simulink library "casper_library_correlator"  (Simulink 8.0)
settings: Solver=ode45  SolverMode=SingleTasking  StartTime=0.0  StopTime=10.0  RelTol=1e-3
values from neighbouring files (symbols this model uses):
  n_bits = eval(get_var('n_bits', 'defaults', defaults, varargin{:}))    [auto_tap_init.m]    (also in baseline_tap_init.m; bi_real_unscr_2x_init.m = get_var('n_bits', 'defaults', defaults, varargin{:}); bi_real_unscr_4x_init.m = get_var('n_bits', 'defaults', defaults, varargin{:}); bit_reverse_init.m = get_var('n_bits',varargin{:}))
libraries: xbsIndex_r4 x1360, casper_library_misc x140, casper_library_multipliers x32, xps_library x8, casper_library_delays x1, casper_library_correlator x1
(part 10 of 14)

== system casper_library_correlator/auto_tap/dual_pol_cmac/cmac1/cmult* ==
  a : Inport
  b : Inport  Port=2
  a_expand : Subsystem  AncestorBlock=casper_library_flow_control/bus_expand  mask(bus_expand){mode=divisions of equal size, outputNum=4, outputWidth=[4 4 4 4], outputBinaryPt=[3 3 3 3], outputArithmeticType=[1 1 1 1], show_format=off, outputToWorkspace=off, variablePrefix=out, outputToModelAsWell=on}
      mask prompts: outputNum "Number of outputs:"; outputWidth "Output width:"; outputBinaryPt "Output binary point position:"; outputArithmeticType "Output arithmetic type (ufix=0, fix=1, bool=2):"; show_format "Print format string?"; outputToWorkspace "Output to workspace?"; variablePrefix "Variable name prefix:"; outputToModelAsWell "Output to model as well?"
      mask help:
      | Expands a 'bus' made using a bus_create or Xilinx
      | concat block.
      | The input will be divided into the specified number
      | of outputs with the specified arithmetic types.
      | Divisions are made from most significant bit.
      mask init: same as casper_library_correlator/dual_pol_cmac/cmac1/cmult*/a_expand
      settings: AttributesFormatString=4 outputs
      mask TypeOptions mode: divisions of equal size | divisions of arbitrary size
      mask Callback mode: bus_expand_callback();
      mask Callback outputWidth: bus_expand_callback();
      mask Callback outputToWorkspace: bus_expand_callback();
  a_replicate : Subsystem  AncestorBlock=casper_library_bus/bus_replicate  mask(bus_replicate){replication=2, latency=0, misc=off, implementation=core}
      mask prompts: replication "replication factor"; misc "misc support"; implementation "delay implementation"
      mask help: Output bus formed by replicating input bus a number of times
      mask init:
      | bus_replicate_init(gcb, ...
      |     'replication', replication, ...
      |     'latency', latency, ...
      |     'implementation', implementation, ...
      |     'misc', misc);
      mask TypeOptions implementation: core | behavioral
  addsub_im : xbsIndex_r4/AddSub  mode=Subtraction  use_carryin=off  use_carryout=off  en=off  latency=1  precision=Full  arith_type=Unsigned  n_bits=16  bin_pt=14  quantization=Truncate  overflow=Wrap  dbl_ovrd=off  use_behavioral_HDL=on  hw_selection=Fabric  pipelined=on  use_rpm=on  block_type=addsub
  addsub_re : xbsIndex_r4/AddSub  mode=Addition  use_carryin=off  use_carryout=off  en=off  latency=1  precision=Full  arith_type=Unsigned  n_bits=16  bin_pt=14  quantization=Truncate  overflow=Wrap  dbl_ovrd=off  use_behavioral_HDL=on  hw_selection=Fabric  pipelined=on  use_rpm=on  block_type=addsub
  b_expand : Subsystem  AncestorBlock=casper_library_flow_control/bus_expand  mask(bus_expand){mode=divisions of equal size, outputNum=4, outputWidth=[4 4 4 4], outputBinaryPt=[3 3 3 3], outputArithmeticType=[1 1 1 1], show_format=off, outputToWorkspace=off, variablePrefix=out, outputToModelAsWell=on}
      mask prompts: outputNum "Number of outputs:"; outputWidth "Output width:"; outputBinaryPt "Output binary point position:"; outputArithmeticType "Output arithmetic type (ufix=0, fix=1, bool=2):"; show_format "Print format string?"; outputToWorkspace "Output to workspace?"; variablePrefix "Variable name prefix:"; outputToModelAsWell "Output to model as well?"
      mask help:
      | Expands a 'bus' made using a bus_create or Xilinx
      | concat block.
      | The input will be divided into the specified number
      | of outputs with the specified arithmetic types.
      | Divisions are made from most significant bit.
      mask init: same as casper_library_correlator/dual_pol_cmac/cmac1/cmult*/a_expand
      settings: AttributesFormatString=4 outputs
      mask TypeOptions mode: divisions of equal size | divisions of arbitrary size
      mask Callback mode: bus_expand_callback();
      mask Callback outputWidth: bus_expand_callback();
      mask Callback outputToWorkspace: bus_expand_callback();
  b_replicate : Subsystem  AncestorBlock=casper_library_bus/bus_replicate  mask(bus_replicate){replication=2, latency=0, misc=off, implementation=core}
      mask prompts: replication "replication factor"; misc "misc support"; implementation "delay implementation"
      mask help: Output bus formed by replicating input bus a number of times
      mask init:
      | bus_replicate_init(gcb, ...
      |     'replication', replication, ...
      |     'latency', latency, ...
      |     'implementation', implementation, ...
      |     'misc', misc);
      mask TypeOptions implementation: core | behavioral
  convert_im : xbsIndex_r4/Convert  gui_display_data_type=Fixed-point  arith_type="Signed  (2's comp)"  n_bits=16  bin_pt=6  float_type=Single  exp_bits=8  fraction_bits=24  quantization=Truncate  overflow=Wrap  en=off  latency=0  dbl_ovrd=off  pipeline=on  block_type=convert
  convert_re : xbsIndex_r4/Convert  gui_display_data_type=Fixed-point  arith_type="Signed  (2's comp)"  n_bits=16  bin_pt=6  float_type=Single  exp_bits=8  fraction_bits=24  quantization=Truncate  overflow=Wrap  en=off  latency=0  dbl_ovrd=off  pipeline=on  block_type=convert
  imim : xbsIndex_r4/Mult  precision=Full  arith_type="Signed  (2's comp)"  n_bits=16  bin_pt=14  quantization=Truncate  overflow=Wrap  en=off  latency=1  dbl_ovrd=off  use_behavioral_HDL=off  opt=Speed  use_embedded=on  optimum_pipeline=off  pipeline=on  use_rpm=on  placement_style=Triangular  block_type=mult
  imre : xbsIndex_r4/Mult  precision=Full  arith_type="Signed  (2's comp)"  n_bits=16  bin_pt=14  quantization=Truncate  overflow=Wrap  en=off  latency=1  dbl_ovrd=off  use_behavioral_HDL=off  opt=Speed  use_embedded=on  optimum_pipeline=off  pipeline=on  use_rpm=on  placement_style=Triangular  block_type=mult
  reim : xbsIndex_r4/Mult  precision=Full  arith_type="Signed  (2's comp)"  n_bits=16  bin_pt=14  quantization=Truncate  overflow=Wrap  en=off  latency=1  dbl_ovrd=off  use_behavioral_HDL=off  opt=Speed  use_embedded=on  optimum_pipeline=off  pipeline=on  use_rpm=on  placement_style=Triangular  block_type=mult
  rere : xbsIndex_r4/Mult  precision=Full  arith_type="Signed  (2's comp)"  n_bits=16  bin_pt=14  quantization=Truncate  overflow=Wrap  en=off  latency=1  dbl_ovrd=off  use_behavioral_HDL=off  opt=Speed  use_embedded=on  optimum_pipeline=off  pipeline=on  use_rpm=on  placement_style=Triangular  block_type=mult
  ri_to_c : casper_library_misc/ri_to_c
  ab : Outport
  wires:
  ri_to_c/1 -> ab/1
  convert_im/1 -> ri_to_c/2
  convert_re/1 -> ri_to_c/1
  addsub_im/1 -> convert_im/1
  addsub_re/1 -> convert_re/1
  reim/1 -> addsub_im/2
  imre/1 -> addsub_im/1
  imim/1 -> addsub_re/2
  rere/1 -> addsub_re/1
  b_expand/4(lsb_out1) -> reim/2
  a_expand/3(out2) -> reim/1
  b_expand/3(out2) -> imre/2
  a_expand/4(lsb_out1) -> imre/1
  b_expand/2(out3) -> imim/2
  a_expand/2(out3) -> imim/1
  b_expand/1(msb_out4) -> rere/2
  a_expand/1(msb_out4) -> rere/1
  b_replicate/1(out) -> b_expand/1(bus_in)
  a_replicate/1(out) -> a_expand/1(bus_in)
  b/1 -> b_replicate/1(in)
  a/1 -> a_replicate/1(in)

== system casper_library_correlator/auto_tap/dual_pol_cmac/cmac1/ri_to_c ==
  In1 : Inport
  In2 : Inport  Port=2
  Concat : xbsIndex_r4/Concat  num_inputs=2  dbl_ovrd=off  block_type=concat
      settings: block_version=9.2.01
  Reinterpret : xbsIndex_r4/Reinterpret  force_arith_type=on  arith_type=Unsigned  force_bin_pt=on  bin_pt=0  block_type=reinterpret
      settings: infoedit="Changes signal type without altering the binary representation.   You can changed the signal between signed and unsigned, and relocate the binary point.<P><P>Hardware notes: In hardware this block costs nothing.<P><P>Example:  Suppose the input is 6 bits wide, signed, with 2 fractional bits, and the output is forced to unsigned with 0 fractional bits.  Then an input of -2.0 (1110.00 in binary 2's complement) becomes an output of 56 (111000 in binary)."  block_version=9.2.01
  Reinterpret1 : xbsIndex_r4/Reinterpret  force_arith_type=on  arith_type=Unsigned  force_bin_pt=on  bin_pt=0  block_type=reinterpret
      settings: infoedit="Changes signal type without altering the binary representation.   You can changed the signal between signed and unsigned, and relocate the binary point.<P><P>Hardware notes: In hardware this block costs nothing.<P><P>Example:  Suppose the input is 6 bits wide, signed, with 2 fractional bits, and the output is forced to unsigned with 0 fractional bits.  Then an input of -2.0 (1110.00 in binary 2's complement) becomes an output of 56 (111000 in binary)."  block_version=9.2.01
  Out1 : Outport
  wires:
  In2/1 -> Reinterpret1/1
  Concat/1 -> Out1/1
  In1/1 -> Reinterpret/1
  Reinterpret1/1 -> Concat/2
  Reinterpret/1 -> Concat/1

== system casper_library_correlator/auto_tap/dual_pol_cmac/cmac2/acc ==
  rst : Inport
  din : Inport  Port=2
  acc_in : Inport  Port=3
  valid_in : Inport  Port=4
  Accumulator : xbsIndex_r4/Accumulator  operation=Add  n_bits=n_bits_out  overflow=Wrap  scale=1  rst=on  infoeditControl=reset for floating point data type must be asserted for a minimum of 2 cycles  hasbypass=on  en=off  latency=0  dbl_ovrd=off  msb_inp=100  msb=100  lsb=-100  use_behavioral_HDL=on  implementation=Fabric  block_type=accum
      settings: infoedit="Adder or subtractor-based accumulator.   Output type and binary point position match the input.<P><P>Hardware notes: When \"Reinitialize with input 'b' on reset\" is selected, the accumulator is forced to run at the system rate even if the input 'b' is running at a slower rate."  xl_area=[0, 0, 0, 0, 0, 0, 0]  block_version=9.2.01
  Constant : xbsIndex_r4/Constant  const=1  gui_display_data_type=Fixed-point  arith_type=Boolean  n_bits=1  bin_pt=0  preci_type=Single  exp_width=8  frac_width=24  explicit_period=on  period=1  equ=P=C  opselect=C  inp2=PCIN>>17  opr=+  inp1=P  carry=CIN  dbl_ovrd=off  block_type=constant
      settings: block_version=9.2.01
  Convert1 : xbsIndex_r4/Convert  gui_display_data_type=Fixed-point  arith_type="Signed  (2's comp)"  n_bits=n_bits_out  bin_pt=bin_pt_out  float_type=Single  exp_bits=8  fraction_bits=24  quantization=Truncate  overflow=Wrap  en=off  latency=0  dbl_ovrd=off  pipeline=off  block_type=convert
      settings: xl_area=[0, 0, 0, 0, 0, 0, 0]  block_version=9.2.01
  Convert2 : xbsIndex_r4/Convert  gui_display_data_type=Fixed-point  arith_type=Boolean  n_bits=8  bin_pt=6  float_type=Single  exp_bits=8  fraction_bits=24  quantization=Truncate  overflow=Wrap  en=off  latency=0  dbl_ovrd=off  pipeline=off  block_type=convert
      settings: xl_area=[0, 0, 0, 0, 0, 0, 0]  block_version=9.2.01
  Delay : xbsIndex_r4/Delay  rst=off  infoeditControl=Selection of Reset will increase slice count due to use of real FFs and instead of SRLs  en=off  latency=0  dbl_ovrd=off  reg_retiming=off  block_type=delay
      settings: xl_area=[0, 0, 0, 0, 0, 0, 0]  block_version=9.2.01
  Delay1 : xbsIndex_r4/Delay  rst=off  infoeditControl=Selection of Reset will increase slice count due to use of real FFs and instead of SRLs  en=off  latency=0  dbl_ovrd=off  reg_retiming=off  block_type=delay
      settings: xl_area=[0, 0, 0, 0, 0, 0, 0]  block_version=9.2.01
  Mux2 : xbsIndex_r4/Mux  inputs=2  en=off  latency=2  precision=Full  arith_type="Signed  (2's comp)"  n_bits=0  bin_pt=0  quantization="Round  (unbiased: +/- Inf)"  overflow=Wrap  dbl_ovrd=off  block_type=mux
      settings: xl_area=[0, 0, 0, 0, 0, 0, 0]  block_version=9.2.01
  Mux3 : xbsIndex_r4/Mux  inputs=2  en=off  latency=2  precision=Full  arith_type="Signed  (2's comp)"  n_bits=0  bin_pt=0  quantization=Truncate  overflow=Wrap  dbl_ovrd=off  block_type=mux
      settings: xl_area=[0, 0, 0, 0, 0, 0, 0]  block_version=9.2.01
  acc_out : Outport
  valid_out : Outport  Port=2
  wires:
  Convert2/1 -> Mux3/2
  Delay1/1 -> Delay/1, Accumulator/2
  Convert1/1 -> Accumulator/1
  Delay/1 -> Mux2/1, Mux3/1
  rst/1 -> Delay1/1
  din/1 -> Convert1/1
  Mux3/1 -> valid_out/1
  Constant/1 -> Mux3/3
  valid_in/1 -> Convert2/1
  acc_in/1 -> Mux2/2
  Mux2/1 -> acc_out/1
  Accumulator/1 -> Mux2/3

== system casper_library_correlator/auto_tap/dual_pol_cmac/cmac2/acc1 ==
  rst : Inport
  din : Inport  Port=2
  acc_in : Inport  Port=3
  valid_in : Inport  Port=4
  Accumulator : xbsIndex_r4/Accumulator  operation=Add  n_bits=n_bits_out  overflow=Wrap  scale=1  rst=on  infoeditControl=reset for floating point data type must be asserted for a minimum of 2 cycles  hasbypass=on  en=off  latency=0  dbl_ovrd=off  msb_inp=100  msb=100  lsb=-100  use_behavioral_HDL=on  implementation=Fabric  block_type=accum
      settings: infoedit="Adder or subtractor-based accumulator.   Output type and binary point position match the input.<P><P>Hardware notes: When \"Reinitialize with input 'b' on reset\" is selected, the accumulator is forced to run at the system rate even if the input 'b' is running at a slower rate."  xl_area=[0, 0, 0, 0, 0, 0, 0]  block_version=9.2.01
  Constant : xbsIndex_r4/Constant  const=1  gui_display_data_type=Fixed-point  arith_type=Boolean  n_bits=1  bin_pt=0  preci_type=Single  exp_width=8  frac_width=24  explicit_period=on  period=1  equ=P=C  opselect=C  inp2=PCIN>>17  opr=+  inp1=P  carry=CIN  dbl_ovrd=off  block_type=constant
      settings: block_version=9.2.01
  Convert1 : xbsIndex_r4/Convert  gui_display_data_type=Fixed-point  arith_type="Signed  (2's comp)"  n_bits=n_bits_out  bin_pt=bin_pt_out  float_type=Single  exp_bits=8  fraction_bits=24  quantization=Truncate  overflow=Wrap  en=off  latency=0  dbl_ovrd=off  pipeline=off  block_type=convert
      settings: xl_area=[0, 0, 0, 0, 0, 0, 0]  block_version=9.2.01
  Convert2 : xbsIndex_r4/Convert  gui_display_data_type=Fixed-point  arith_type=Boolean  n_bits=8  bin_pt=6  float_type=Single  exp_bits=8  fraction_bits=24  quantization=Truncate  overflow=Wrap  en=off  latency=0  dbl_ovrd=off  pipeline=off  block_type=convert
      settings: xl_area=[0, 0, 0, 0, 0, 0, 0]  block_version=9.2.01
  Delay : xbsIndex_r4/Delay  rst=off  infoeditControl=Selection of Reset will increase slice count due to use of real FFs and instead of SRLs  en=off  latency=0  dbl_ovrd=off  reg_retiming=off  block_type=delay
      settings: xl_area=[0, 0, 0, 0, 0, 0, 0]  block_version=9.2.01
  Delay1 : xbsIndex_r4/Delay  rst=off  infoeditControl=Selection of Reset will increase slice count due to use of real FFs and instead of SRLs  en=off  latency=0  dbl_ovrd=off  reg_retiming=off  block_type=delay
      settings: xl_area=[0, 0, 0, 0, 0, 0, 0]  block_version=9.2.01
  Mux2 : xbsIndex_r4/Mux  inputs=2  en=off  latency=2  precision=Full  arith_type="Signed  (2's comp)"  n_bits=0  bin_pt=0  quantization="Round  (unbiased: +/- Inf)"  overflow=Wrap  dbl_ovrd=off  block_type=mux
      settings: xl_area=[0, 0, 0, 0, 0, 0, 0]  block_version=9.2.01
  Mux3 : xbsIndex_r4/Mux  inputs=2  en=off  latency=2  precision=Full  arith_type="Signed  (2's comp)"  n_bits=0  bin_pt=0  quantization=Truncate  overflow=Wrap  dbl_ovrd=off  block_type=mux
      settings: xl_area=[0, 0, 0, 0, 0, 0, 0]  block_version=9.2.01
  acc_out : Outport
  valid_out : Outport  Port=2
  wires:
  Accumulator/1 -> Mux2/3
  Mux2/1 -> acc_out/1
  acc_in/1 -> Mux2/2
  valid_in/1 -> Convert2/1
  Constant/1 -> Mux3/3
  Mux3/1 -> valid_out/1
  din/1 -> Convert1/1
  rst/1 -> Delay1/1
  Delay/1 -> Mux3/1, Mux2/1
  Convert1/1 -> Accumulator/1
  Delay1/1 -> Accumulator/2, Delay/1
  Convert2/1 -> Mux3/2

== system casper_library_correlator/auto_tap/dual_pol_cmac/cmac2/c_to_ri1 ==
  In1 : Inport
  Reinterpret : xbsIndex_r4/Reinterpret  force_arith_type=on  arith_type="Signed  (2's comp)"  force_bin_pt=on  bin_pt=bin_pt_out  block_type=reinterpret
      settings: block_version=9.2.01
  Reinterpret1 : xbsIndex_r4/Reinterpret  force_arith_type=on  arith_type="Signed  (2's comp)"  force_bin_pt=on  bin_pt=bin_pt_out  block_type=reinterpret
      settings: block_version=9.2.01
  Slice : xbsIndex_r4/Slice  nbits=n_bits_out  boolean_output=off  mode=Upper Bit Location + Width  bit1=0  base1=MSB of Input  bit0=0  base0=LSB of Input  dbl_ovrd=off  block_type=slice
      settings: infoedit="Extracts a given range of bits from each input sample and presents it at the output.  The output type is ordinarily unsigned with binary point at zero, but can be Boolean when the slice is one bit wide.<P><P>Hardware notes: In hardware this block costs nothing."  block_version=9.2.01
  Slice1 : xbsIndex_r4/Slice  nbits=n_bits_out  boolean_output=off  mode=Lower Bit Location + Width  bit1=0  base1=MSB of Input  bit0=0  base0=LSB of Input  dbl_ovrd=off  block_type=slice
      settings: infoedit="Extracts a given range of bits from each input sample and presents it at the output.  The output type is ordinarily unsigned with binary point at zero, but can be Boolean when the slice is one bit wide.<P><P>Hardware notes: In hardware this block costs nothing."  block_version=9.2.01
  Out1 : Outport
  Out2 : Outport  Port=2
  wires:
  In1/1 -> Slice1/1, Slice/1
  Reinterpret1/1 -> Out2/1
  Reinterpret/1 -> Out1/1
  Slice1/1 -> Reinterpret1/1
  Slice/1 -> Reinterpret/1

== system casper_library_correlator/auto_tap/dual_pol_cmac/cmac2/c_to_ri2 ==
  In1 : Inport
  Reinterpret : xbsIndex_r4/Reinterpret  force_arith_type=on  arith_type="Signed  (2's comp)"  force_bin_pt=on  bin_pt=n_bits_out - bit_growth - 3  block_type=reinterpret
      settings: infoedit="Changes signal type without altering the binary representation.   You can changed the signal between signed and unsigned, and relocate the binary point.<P><P>Hardware notes: In hardware this block costs nothing.<P><P>Example:  Suppose the input is 6 bits wide, signed, with 2 fractional bits, and the output is forced to unsigned with 0 fractional bits.  Then an input of -2.0 (1110.00 in binary 2's complement) becomes an output of 56 (111000 in binary)."  block_version=9.2.01
  Reinterpret1 : xbsIndex_r4/Reinterpret  force_arith_type=on  arith_type="Signed  (2's comp)"  force_bin_pt=on  bin_pt=n_bits_out - bit_growth - 3  block_type=reinterpret
      settings: infoedit="Changes signal type without altering the binary representation.   You can changed the signal between signed and unsigned, and relocate the binary point.<P><P>Hardware notes: In hardware this block costs nothing.<P><P>Example:  Suppose the input is 6 bits wide, signed, with 2 fractional bits, and the output is forced to unsigned with 0 fractional bits.  Then an input of -2.0 (1110.00 in binary 2's complement) becomes an output of 56 (111000 in binary)."  block_version=9.2.01
  Slice : xbsIndex_r4/Slice  nbits=n_bits_out  boolean_output=off  mode=Upper Bit Location + Width  bit1=0  base1=MSB of Input  bit0=0  base0=LSB of Input  dbl_ovrd=off  block_type=slice
      settings: infoedit="Extracts a given range of bits from each input sample and presents it at the output.  The output type is ordinarily unsigned with binary point at zero, but can be Boolean when the slice is one bit wide.<P><P>Hardware notes: In hardware this block costs nothing."  block_version=9.2.01
  Slice1 : xbsIndex_r4/Slice  nbits=n_bits_out  boolean_output=off  mode=Lower Bit Location + Width  bit1=0  base1=MSB of Input  bit0=0  base0=LSB of Input  dbl_ovrd=off  block_type=slice
      settings: infoedit="Extracts a given range of bits from each input sample and presents it at the output.  The output type is ordinarily unsigned with binary point at zero, but can be Boolean when the slice is one bit wide.<P><P>Hardware notes: In hardware this block costs nothing."  block_version=9.2.01
  Out1 : Outport
  Out2 : Outport  Port=2
  wires:
  Slice/1 -> Reinterpret/1
  Slice1/1 -> Reinterpret1/1
  Reinterpret/1 -> Out1/1
  Reinterpret1/1 -> Out2/1
  In1/1 -> Slice/1, Slice1/1

== system casper_library_correlator/auto_tap/dual_pol_cmac/cmac2/cmult* ==
  a : Inport
  b : Inport  Port=2
  a_expand : Subsystem  AncestorBlock=casper_library_flow_control/bus_expand  mask(bus_expand){mode=divisions of equal size, outputNum=4, outputWidth=[4 4 4 4], outputBinaryPt=[3 3 3 3], outputArithmeticType=[1 1 1 1], show_format=off, outputToWorkspace=off, variablePrefix=out, outputToModelAsWell=on}
      mask prompts: outputNum "Number of outputs:"; outputWidth "Output width:"; outputBinaryPt "Output binary point position:"; outputArithmeticType "Output arithmetic type (ufix=0, fix=1, bool=2):"; show_format "Print format string?"; outputToWorkspace "Output to workspace?"; variablePrefix "Variable name prefix:"; outputToModelAsWell "Output to model as well?"
      mask help:
      | Expands a 'bus' made using a bus_create or Xilinx
      | concat block.
      | The input will be divided into the specified number
      | of outputs with the specified arithmetic types.
      | Divisions are made from most significant bit.
      mask init: same as casper_library_correlator/dual_pol_cmac/cmac1/cmult*/a_expand
      settings: AttributesFormatString=4 outputs
      mask TypeOptions mode: divisions of equal size | divisions of arbitrary size
      mask Callback mode: bus_expand_callback();
      mask Callback outputWidth: bus_expand_callback();
      mask Callback outputToWorkspace: bus_expand_callback();
  a_replicate : Subsystem  AncestorBlock=casper_library_bus/bus_replicate  mask(bus_replicate){replication=2, latency=0, misc=off, implementation=core}
      mask prompts: replication "replication factor"; misc "misc support"; implementation "delay implementation"
      mask help: Output bus formed by replicating input bus a number of times
      mask init:
      | bus_replicate_init(gcb, ...
      |     'replication', replication, ...
      |     'latency', latency, ...
      |     'implementation', implementation, ...
      |     'misc', misc);
      mask TypeOptions implementation: core | behavioral
  addsub_im : xbsIndex_r4/AddSub  mode=Subtraction  use_carryin=off  use_carryout=off  en=off  latency=1  precision=Full  arith_type=Unsigned  n_bits=16  bin_pt=14  quantization=Truncate  overflow=Wrap  dbl_ovrd=off  use_behavioral_HDL=on  hw_selection=Fabric  pipelined=on  use_rpm=on  block_type=addsub
  addsub_re : xbsIndex_r4/AddSub  mode=Addition  use_carryin=off  use_carryout=off  en=off  latency=1  precision=Full  arith_type=Unsigned  n_bits=16  bin_pt=14  quantization=Truncate  overflow=Wrap  dbl_ovrd=off  use_behavioral_HDL=on  hw_selection=Fabric  pipelined=on  use_rpm=on  block_type=addsub
  b_expand : Subsystem  AncestorBlock=casper_library_flow_control/bus_expand  mask(bus_expand){mode=divisions of equal size, outputNum=4, outputWidth=[4 4 4 4], outputBinaryPt=[3 3 3 3], outputArithmeticType=[1 1 1 1], show_format=off, outputToWorkspace=off, variablePrefix=out, outputToModelAsWell=on}
      mask prompts: outputNum "Number of outputs:"; outputWidth "Output width:"; outputBinaryPt "Output binary point position:"; outputArithmeticType "Output arithmetic type (ufix=0, fix=1, bool=2):"; show_format "Print format string?"; outputToWorkspace "Output to workspace?"; variablePrefix "Variable name prefix:"; outputToModelAsWell "Output to model as well?"
      mask help:
      | Expands a 'bus' made using a bus_create or Xilinx
      | concat block.
      | The input will be divided into the specified number
      | of outputs with the specified arithmetic types.
      | Divisions are made from most significant bit.
      mask init: same as casper_library_correlator/dual_pol_cmac/cmac1/cmult*/a_expand
      settings: AttributesFormatString=4 outputs
      mask TypeOptions mode: divisions of equal size | divisions of arbitrary size
      mask Callback mode: bus_expand_callback();
      mask Callback outputWidth: bus_expand_callback();
      mask Callback outputToWorkspace: bus_expand_callback();
  b_replicate : Subsystem  AncestorBlock=casper_library_bus/bus_replicate  mask(bus_replicate){replication=2, latency=0, misc=off, implementation=core}
      mask prompts: replication "replication factor"; misc "misc support"; implementation "delay implementation"
      mask help: Output bus formed by replicating input bus a number of times
      mask init:
      | bus_replicate_init(gcb, ...
      |     'replication', replication, ...
      |     'latency', latency, ...
      |     'implementation', implementation, ...
      |     'misc', misc);
      mask TypeOptions implementation: core | behavioral
  convert_im : xbsIndex_r4/Convert  gui_display_data_type=Fixed-point  arith_type="Signed  (2's comp)"  n_bits=16  bin_pt=6  float_type=Single  exp_bits=8  fraction_bits=24  quantization=Truncate  overflow=Wrap  en=off  latency=0  dbl_ovrd=off  pipeline=on  block_type=convert
  convert_re : xbsIndex_r4/Convert  gui_display_data_type=Fixed-point  arith_type="Signed  (2's comp)"  n_bits=16  bin_pt=6  float_type=Single  exp_bits=8  fraction_bits=24  quantization=Truncate  overflow=Wrap  en=off  latency=0  dbl_ovrd=off  pipeline=on  block_type=convert
  imim : xbsIndex_r4/Mult  precision=Full  arith_type="Signed  (2's comp)"  n_bits=16  bin_pt=14  quantization=Truncate  overflow=Wrap  en=off  latency=1  dbl_ovrd=off  use_behavioral_HDL=off  opt=Speed  use_embedded=on  optimum_pipeline=off  pipeline=on  use_rpm=on  placement_style=Triangular  block_type=mult
  imre : xbsIndex_r4/Mult  precision=Full  arith_type="Signed  (2's comp)"  n_bits=16  bin_pt=14  quantization=Truncate  overflow=Wrap  en=off  latency=1  dbl_ovrd=off  use_behavioral_HDL=off  opt=Speed  use_embedded=on  optimum_pipeline=off  pipeline=on  use_rpm=on  placement_style=Triangular  block_type=mult
  reim : xbsIndex_r4/Mult  precision=Full  arith_type="Signed  (2's comp)"  n_bits=16  bin_pt=14  quantization=Truncate  overflow=Wrap  en=off  latency=1  dbl_ovrd=off  use_behavioral_HDL=off  opt=Speed  use_embedded=on  optimum_pipeline=off  pipeline=on  use_rpm=on  placement_style=Triangular  block_type=mult
  rere : xbsIndex_r4/Mult  precision=Full  arith_type="Signed  (2's comp)"  n_bits=16  bin_pt=14  quantization=Truncate  overflow=Wrap  en=off  latency=1  dbl_ovrd=off  use_behavioral_HDL=off  opt=Speed  use_embedded=on  optimum_pipeline=off  pipeline=on  use_rpm=on  placement_style=Triangular  block_type=mult
  ri_to_c : casper_library_misc/ri_to_c
  ab : Outport
  wires:
  ri_to_c/1 -> ab/1
  convert_im/1 -> ri_to_c/2
  convert_re/1 -> ri_to_c/1
  addsub_im/1 -> convert_im/1
  addsub_re/1 -> convert_re/1
  reim/1 -> addsub_im/2
  imre/1 -> addsub_im/1
  imim/1 -> addsub_re/2
  rere/1 -> addsub_re/1
  b_expand/4(lsb_out1) -> reim/2
  a_expand/3(out2) -> reim/1
  b_expand/3(out2) -> imre/2
  a_expand/4(lsb_out1) -> imre/1
  b_expand/2(out3) -> imim/2
  a_expand/2(out3) -> imim/1
  b_expand/1(msb_out4) -> rere/2
  a_expand/1(msb_out4) -> rere/1
  b_replicate/1(out) -> b_expand/1(bus_in)
  a_replicate/1(out) -> a_expand/1(bus_in)
  b/1 -> b_replicate/1(in)
  a/1 -> a_replicate/1(in)

== system casper_library_correlator/auto_tap/dual_pol_cmac/cmac2/ri_to_c ==
  In1 : Inport
  In2 : Inport  Port=2
  Concat : xbsIndex_r4/Concat  num_inputs=2  dbl_ovrd=off  block_type=concat
      settings: block_version=9.2.01
  Reinterpret : xbsIndex_r4/Reinterpret  force_arith_type=on  arith_type=Unsigned  force_bin_pt=on  bin_pt=0  block_type=reinterpret
      settings: infoedit="Changes signal type without altering the binary representation.   You can changed the signal between signed and unsigned, and relocate the binary point.<P><P>Hardware notes: In hardware this block costs nothing.<P><P>Example:  Suppose the input is 6 bits wide, signed, with 2 fractional bits, and the output is forced to unsigned with 0 fractional bits.  Then an input of -2.0 (1110.00 in binary 2's complement) becomes an output of 56 (111000 in binary)."  block_version=9.2.01
  Reinterpret1 : xbsIndex_r4/Reinterpret  force_arith_type=on  arith_type=Unsigned  force_bin_pt=on  bin_pt=0  block_type=reinterpret
      settings: infoedit="Changes signal type without altering the binary representation.   You can changed the signal between signed and unsigned, and relocate the binary point.<P><P>Hardware notes: In hardware this block costs nothing.<P><P>Example:  Suppose the input is 6 bits wide, signed, with 2 fractional bits, and the output is forced to unsigned with 0 fractional bits.  Then an input of -2.0 (1110.00 in binary 2's complement) becomes an output of 56 (111000 in binary)."  block_version=9.2.01
  Out1 : Outport
  wires:
  In2/1 -> Reinterpret1/1
  Concat/1 -> Out1/1
  In1/1 -> Reinterpret/1
  Reinterpret1/1 -> Concat/2
  Reinterpret/1 -> Concat/1

== system casper_library_correlator/auto_tap/dual_pol_cmac/cmac3/acc ==
  rst : Inport
  din : Inport  Port=2
  acc_in : Inport  Port=3
  valid_in : Inport  Port=4
  Accumulator : xbsIndex_r4/Accumulator  operation=Add  n_bits=n_bits_out  overflow=Wrap  scale=1  rst=on  infoeditControl=reset for floating point data type must be asserted for a minimum of 2 cycles  hasbypass=on  en=off  latency=0  dbl_ovrd=off  msb_inp=100  msb=100  lsb=-100  use_behavioral_HDL=on  implementation=Fabric  block_type=accum
      settings: infoedit="Adder or subtractor-based accumulator.   Output type and binary point position match the input.<P><P>Hardware notes: When \"Reinitialize with input 'b' on reset\" is selected, the accumulator is forced to run at the system rate even if the input 'b' is running at a slower rate."  xl_area=[0, 0, 0, 0, 0, 0, 0]  block_version=9.2.01
  Constant : xbsIndex_r4/Constant  const=1  gui_display_data_type=Fixed-point  arith_type=Boolean  n_bits=1  bin_pt=0  preci_type=Single  exp_width=8  frac_width=24  explicit_period=on  period=1  equ=P=C  opselect=C  inp2=PCIN>>17  opr=+  inp1=P  carry=CIN  dbl_ovrd=off  block_type=constant
      settings: block_version=9.2.01
  Convert1 : xbsIndex_r4/Convert  gui_display_data_type=Fixed-point  arith_type="Signed  (2's comp)"  n_bits=n_bits_out  bin_pt=bin_pt_out  float_type=Single  exp_bits=8  fraction_bits=24  quantization=Truncate  overflow=Wrap  en=off  latency=0  dbl_ovrd=off  pipeline=off  block_type=convert
      settings: xl_area=[0, 0, 0, 0, 0, 0, 0]  block_version=9.2.01
  Convert2 : xbsIndex_r4/Convert  gui_display_data_type=Fixed-point  arith_type=Boolean  n_bits=8  bin_pt=6  float_type=Single  exp_bits=8  fraction_bits=24  quantization=Truncate  overflow=Wrap  en=off  latency=0  dbl_ovrd=off  pipeline=off  block_type=convert
      settings: xl_area=[0, 0, 0, 0, 0, 0, 0]  block_version=9.2.01
  Delay : xbsIndex_r4/Delay  rst=off  infoeditControl=Selection of Reset will increase slice count due to use of real FFs and instead of SRLs  en=off  latency=0  dbl_ovrd=off  reg_retiming=off  block_type=delay
      settings: xl_area=[0, 0, 0, 0, 0, 0, 0]  block_version=9.2.01
  Delay1 : xbsIndex_r4/Delay  rst=off  infoeditControl=Selection of Reset will increase slice count due to use of real FFs and instead of SRLs  en=off  latency=0  dbl_ovrd=off  reg_retiming=off  block_type=delay
      settings: xl_area=[0, 0, 0, 0, 0, 0, 0]  block_version=9.2.01
  Mux2 : xbsIndex_r4/Mux  inputs=2  en=off  latency=2  precision=Full  arith_type="Signed  (2's comp)"  n_bits=0  bin_pt=0  quantization="Round  (unbiased: +/- Inf)"  overflow=Wrap  dbl_ovrd=off  block_type=mux
      settings: xl_area=[0, 0, 0, 0, 0, 0, 0]  block_version=9.2.01
  Mux3 : xbsIndex_r4/Mux  inputs=2  en=off  latency=2  precision=Full  arith_type="Signed  (2's comp)"  n_bits=0  bin_pt=0  quantization=Truncate  overflow=Wrap  dbl_ovrd=off  block_type=mux
      settings: xl_area=[0, 0, 0, 0, 0, 0, 0]  block_version=9.2.01
  acc_out : Outport
  valid_out : Outport  Port=2
  wires:
  Convert2/1 -> Mux3/2
  Delay1/1 -> Delay/1, Accumulator/2
  Convert1/1 -> Accumulator/1
  Delay/1 -> Mux2/1, Mux3/1
  rst/1 -> Delay1/1
  din/1 -> Convert1/1
  Mux3/1 -> valid_out/1
  Constant/1 -> Mux3/3
  valid_in/1 -> Convert2/1
  acc_in/1 -> Mux2/2
  Mux2/1 -> acc_out/1
  Accumulator/1 -> Mux2/3

== system casper_library_correlator/auto_tap/dual_pol_cmac/cmac3/acc1 ==
  rst : Inport
  din : Inport  Port=2
  acc_in : Inport  Port=3
  valid_in : Inport  Port=4
  Accumulator : xbsIndex_r4/Accumulator  operation=Add  n_bits=n_bits_out  overflow=Wrap  scale=1  rst=on  infoeditControl=reset for floating point data type must be asserted for a minimum of 2 cycles  hasbypass=on  en=off  latency=0  dbl_ovrd=off  msb_inp=100  msb=100  lsb=-100  use_behavioral_HDL=on  implementation=Fabric  block_type=accum
      settings: infoedit="Adder or subtractor-based accumulator.   Output type and binary point position match the input.<P><P>Hardware notes: When \"Reinitialize with input 'b' on reset\" is selected, the accumulator is forced to run at the system rate even if the input 'b' is running at a slower rate."  xl_area=[0, 0, 0, 0, 0, 0, 0]  block_version=9.2.01
  Constant : xbsIndex_r4/Constant  const=1  gui_display_data_type=Fixed-point  arith_type=Boolean  n_bits=1  bin_pt=0  preci_type=Single  exp_width=8  frac_width=24  explicit_period=on  period=1  equ=P=C  opselect=C  inp2=PCIN>>17  opr=+  inp1=P  carry=CIN  dbl_ovrd=off  block_type=constant
      settings: block_version=9.2.01
  Convert1 : xbsIndex_r4/Convert  gui_display_data_type=Fixed-point  arith_type="Signed  (2's comp)"  n_bits=n_bits_out  bin_pt=bin_pt_out  float_type=Single  exp_bits=8  fraction_bits=24  quantization=Truncate  overflow=Wrap  en=off  latency=0  dbl_ovrd=off  pipeline=off  block_type=convert
      settings: xl_area=[0, 0, 0, 0, 0, 0, 0]  block_version=9.2.01
  Convert2 : xbsIndex_r4/Convert  gui_display_data_type=Fixed-point  arith_type=Boolean  n_bits=8  bin_pt=6  float_type=Single  exp_bits=8  fraction_bits=24  quantization=Truncate  overflow=Wrap  en=off  latency=0  dbl_ovrd=off  pipeline=off  block_type=convert
      settings: xl_area=[0, 0, 0, 0, 0, 0, 0]  block_version=9.2.01
  Delay : xbsIndex_r4/Delay  rst=off  infoeditControl=Selection of Reset will increase slice count due to use of real FFs and instead of SRLs  en=off  latency=0  dbl_ovrd=off  reg_retiming=off  block_type=delay
      settings: xl_area=[0, 0, 0, 0, 0, 0, 0]  block_version=9.2.01
  Delay1 : xbsIndex_r4/Delay  rst=off  infoeditControl=Selection of Reset will increase slice count due to use of real FFs and instead of SRLs  en=off  latency=0  dbl_ovrd=off  reg_retiming=off  block_type=delay
      settings: xl_area=[0, 0, 0, 0, 0, 0, 0]  block_version=9.2.01
  Mux2 : xbsIndex_r4/Mux  inputs=2  en=off  latency=2  precision=Full  arith_type="Signed  (2's comp)"  n_bits=0  bin_pt=0  quantization="Round  (unbiased: +/- Inf)"  overflow=Wrap  dbl_ovrd=off  block_type=mux
      settings: xl_area=[0, 0, 0, 0, 0, 0, 0]  block_version=9.2.01
  Mux3 : xbsIndex_r4/Mux  inputs=2  en=off  latency=2  precision=Full  arith_type="Signed  (2's comp)"  n_bits=0  bin_pt=0  quantization=Truncate  overflow=Wrap  dbl_ovrd=off  block_type=mux
      settings: xl_area=[0, 0, 0, 0, 0, 0, 0]  block_version=9.2.01
  acc_out : Outport
  valid_out : Outport  Port=2
  wires:
  Accumulator/1 -> Mux2/3
  Mux2/1 -> acc_out/1
  acc_in/1 -> Mux2/2
  valid_in/1 -> Convert2/1
  Constant/1 -> Mux3/3
  Mux3/1 -> valid_out/1
  din/1 -> Convert1/1
  rst/1 -> Delay1/1
  Delay/1 -> Mux3/1, Mux2/1
  Convert1/1 -> Accumulator/1
  Delay1/1 -> Accumulator/2, Delay/1
  Convert2/1 -> Mux3/2

== system casper_library_correlator/auto_tap/dual_pol_cmac/cmac3/c_to_ri1 ==
  In1 : Inport
  Reinterpret : xbsIndex_r4/Reinterpret  force_arith_type=on  arith_type="Signed  (2's comp)"  force_bin_pt=on  bin_pt=bin_pt_out  block_type=reinterpret
      settings: block_version=9.2.01
  Reinterpret1 : xbsIndex_r4/Reinterpret  force_arith_type=on  arith_type="Signed  (2's comp)"  force_bin_pt=on  bin_pt=bin_pt_out  block_type=reinterpret
      settings: block_version=9.2.01
  Slice : xbsIndex_r4/Slice  nbits=n_bits_out  boolean_output=off  mode=Upper Bit Location + Width  bit1=0  base1=MSB of Input  bit0=0  base0=LSB of Input  dbl_ovrd=off  block_type=slice
      settings: infoedit="Extracts a given range of bits from each input sample and presents it at the output.  The output type is ordinarily unsigned with binary point at zero, but can be Boolean when the slice is one bit wide.<P><P>Hardware notes: In hardware this block costs nothing."  block_version=9.2.01
  Slice1 : xbsIndex_r4/Slice  nbits=n_bits_out  boolean_output=off  mode=Lower Bit Location + Width  bit1=0  base1=MSB of Input  bit0=0  base0=LSB of Input  dbl_ovrd=off  block_type=slice
      settings: infoedit="Extracts a given range of bits from each input sample and presents it at the output.  The output type is ordinarily unsigned with binary point at zero, but can be Boolean when the slice is one bit wide.<P><P>Hardware notes: In hardware this block costs nothing."  block_version=9.2.01
  Out1 : Outport
  Out2 : Outport  Port=2
  wires:
  In1/1 -> Slice1/1, Slice/1
  Reinterpret1/1 -> Out2/1
  Reinterpret/1 -> Out1/1
  Slice1/1 -> Reinterpret1/1
  Slice/1 -> Reinterpret/1

== system casper_library_correlator/auto_tap/dual_pol_cmac/cmac3/c_to_ri2 ==
  In1 : Inport
  Reinterpret : xbsIndex_r4/Reinterpret  force_arith_type=on  arith_type="Signed  (2's comp)"  force_bin_pt=on  bin_pt=n_bits_out - bit_growth - 3  block_type=reinterpret
      settings: infoedit="Changes signal type without altering the binary representation.   You can changed the signal between signed and unsigned, and relocate the binary point.<P><P>Hardware notes: In hardware this block costs nothing.<P><P>Example:  Suppose the input is 6 bits wide, signed, with 2 fractional bits, and the output is forced to unsigned with 0 fractional bits.  Then an input of -2.0 (1110.00 in binary 2's complement) becomes an output of 56 (111000 in binary)."  block_version=9.2.01
  Reinterpret1 : xbsIndex_r4/Reinterpret  force_arith_type=on  arith_type="Signed  (2's comp)"  force_bin_pt=on  bin_pt=n_bits_out - bit_growth - 3  block_type=reinterpret
      settings: infoedit="Changes signal type without altering the binary representation.   You can changed the signal between signed and unsigned, and relocate the binary point.<P><P>Hardware notes: In hardware this block costs nothing.<P><P>Example:  Suppose the input is 6 bits wide, signed, with 2 fractional bits, and the output is forced to unsigned with 0 fractional bits.  Then an input of -2.0 (1110.00 in binary 2's complement) becomes an output of 56 (111000 in binary)."  block_version=9.2.01
  Slice : xbsIndex_r4/Slice  nbits=n_bits_out  boolean_output=off  mode=Upper Bit Location + Width  bit1=0  base1=MSB of Input  bit0=0  base0=LSB of Input  dbl_ovrd=off  block_type=slice
      settings: infoedit="Extracts a given range of bits from each input sample and presents it at the output.  The output type is ordinarily unsigned with binary point at zero, but can be Boolean when the slice is one bit wide.<P><P>Hardware notes: In hardware this block costs nothing."  block_version=9.2.01
  Slice1 : xbsIndex_r4/Slice  nbits=n_bits_out  boolean_output=off  mode=Lower Bit Location + Width  bit1=0  base1=MSB of Input  bit0=0  base0=LSB of Input  dbl_ovrd=off  block_type=slice
      settings: infoedit="Extracts a given range of bits from each input sample and presents it at the output.  The output type is ordinarily unsigned with binary point at zero, but can be Boolean when the slice is one bit wide.<P><P>Hardware notes: In hardware this block costs nothing."  block_version=9.2.01
  Out1 : Outport
  Out2 : Outport  Port=2
  wires:
  Slice/1 -> Reinterpret/1
  Slice1/1 -> Reinterpret1/1
  Reinterpret/1 -> Out1/1
  Reinterpret1/1 -> Out2/1
  In1/1 -> Slice/1, Slice1/1

== system casper_library_correlator/auto_tap/dual_pol_cmac/cmac3/cmult* ==
  a : Inport
  b : Inport  Port=2
  a_expand : Subsystem  AncestorBlock=casper_library_flow_control/bus_expand  mask(bus_expand){mode=divisions of equal size, outputNum=4, outputWidth=[4 4 4 4], outputBinaryPt=[3 3 3 3], outputArithmeticType=[1 1 1 1], show_format=off, outputToWorkspace=off, variablePrefix=out, outputToModelAsWell=on}
      mask prompts: outputNum "Number of outputs:"; outputWidth "Output width:"; outputBinaryPt "Output binary point position:"; outputArithmeticType "Output arithmetic type (ufix=0, fix=1, bool=2):"; show_format "Print format string?"; outputToWorkspace "Output to workspace?"; variablePrefix "Variable name prefix:"; outputToModelAsWell "Output to model as well?"
      mask help:
      | Expands a 'bus' made using a bus_create or Xilinx
      | concat block.
      | The input will be divided into the specified number
      | of outputs with the specified arithmetic types.
      | Divisions are made from most significant bit.
      mask init: same as casper_library_correlator/dual_pol_cmac/cmac1/cmult*/a_expand
      settings: AttributesFormatString=4 outputs
      mask TypeOptions mode: divisions of equal size | divisions of arbitrary size
      mask Callback mode: bus_expand_callback();
      mask Callback outputWidth: bus_expand_callback();
      mask Callback outputToWorkspace: bus_expand_callback();
  a_replicate : Subsystem  AncestorBlock=casper_library_bus/bus_replicate  mask(bus_replicate){replication=2, latency=0, misc=off, implementation=core}
      mask prompts: replication "replication factor"; misc "misc support"; implementation "delay implementation"
      mask help: Output bus formed by replicating input bus a number of times
      mask init:
      | bus_replicate_init(gcb, ...
      |     'replication', replication, ...
      |     'latency', latency, ...
      |     'implementation', implementation, ...
      |     'misc', misc);
      mask TypeOptions implementation: core | behavioral
  addsub_im : xbsIndex_r4/AddSub  mode=Subtraction  use_carryin=off  use_carryout=off  en=off  latency=1  precision=Full  arith_type=Unsigned  n_bits=16  bin_pt=14  quantization=Truncate  overflow=Wrap  dbl_ovrd=off  use_behavioral_HDL=on  hw_selection=Fabric  pipelined=on  use_rpm=on  block_type=addsub
  addsub_re : xbsIndex_r4/AddSub  mode=Addition  use_carryin=off  use_carryout=off  en=off  latency=1  precision=Full  arith_type=Unsigned  n_bits=16  bin_pt=14  quantization=Truncate  overflow=Wrap  dbl_ovrd=off  use_behavioral_HDL=on  hw_selection=Fabric  pipelined=on  use_rpm=on  block_type=addsub
  b_expand : Subsystem  AncestorBlock=casper_library_flow_control/bus_expand  mask(bus_expand){mode=divisions of equal size, outputNum=4, outputWidth=[4 4 4 4], outputBinaryPt=[3 3 3 3], outputArithmeticType=[1 1 1 1], show_format=off, outputToWorkspace=off, variablePrefix=out, outputToModelAsWell=on}
      mask prompts: outputNum "Number of outputs:"; outputWidth "Output width:"; outputBinaryPt "Output binary point position:"; outputArithmeticType "Output arithmetic type (ufix=0, fix=1, bool=2):"; show_format "Print format string?"; outputToWorkspace "Output to workspace?"; variablePrefix "Variable name prefix:"; outputToModelAsWell "Output to model as well?"
      mask help:
      | Expands a 'bus' made using a bus_create or Xilinx
      | concat block.
      | The input will be divided into the specified number
      | of outputs with the specified arithmetic types.
      | Divisions are made from most significant bit.
      mask init: same as casper_library_correlator/dual_pol_cmac/cmac1/cmult*/a_expand
      settings: AttributesFormatString=4 outputs
      mask TypeOptions mode: divisions of equal size | divisions of arbitrary size
      mask Callback mode: bus_expand_callback();
      mask Callback outputWidth: bus_expand_callback();
      mask Callback outputToWorkspace: bus_expand_callback();
  b_replicate : Subsystem  AncestorBlock=casper_library_bus/bus_replicate  mask(bus_replicate){replication=2, latency=0, misc=off, implementation=core}
      mask prompts: replication "replication factor"; misc "misc support"; implementation "delay implementation"
      mask help: Output bus formed by replicating input bus a number of times
      mask init:
      | bus_replicate_init(gcb, ...
      |     'replication', replication, ...
      |     'latency', latency, ...
      |     'implementation', implementation, ...
      |     'misc', misc);
      mask TypeOptions implementation: core | behavioral
  convert_im : xbsIndex_r4/Convert  gui_display_data_type=Fixed-point  arith_type="Signed  (2's comp)"  n_bits=16  bin_pt=6  float_type=Single  exp_bits=8  fraction_bits=24  quantization=Truncate  overflow=Wrap  en=off  latency=0  dbl_ovrd=off  pipeline=on  block_type=convert
  convert_re : xbsIndex_r4/Convert  gui_display_data_type=Fixed-point  arith_type="Signed  (2's comp)"  n_bits=16  bin_pt=6  float_type=Single  exp_bits=8  fraction_bits=24  quantization=Truncate  overflow=Wrap  en=off  latency=0  dbl_ovrd=off  pipeline=on  block_type=convert
  imim : xbsIndex_r4/Mult  precision=Full  arith_type="Signed  (2's comp)"  n_bits=16  bin_pt=14  quantization=Truncate  overflow=Wrap  en=off  latency=1  dbl_ovrd=off  use_behavioral_HDL=off  opt=Speed  use_embedded=on  optimum_pipeline=off  pipeline=on  use_rpm=on  placement_style=Triangular  block_type=mult
  imre : xbsIndex_r4/Mult  precision=Full  arith_type="Signed  (2's comp)"  n_bits=16  bin_pt=14  quantization=Truncate  overflow=Wrap  en=off  latency=1  dbl_ovrd=off  use_behavioral_HDL=off  opt=Speed  use_embedded=on  optimum_pipeline=off  pipeline=on  use_rpm=on  placement_style=Triangular  block_type=mult
  reim : xbsIndex_r4/Mult  precision=Full  arith_type="Signed  (2's comp)"  n_bits=16  bin_pt=14  quantization=Truncate  overflow=Wrap  en=off  latency=1  dbl_ovrd=off  use_behavioral_HDL=off  opt=Speed  use_embedded=on  optimum_pipeline=off  pipeline=on  use_rpm=on  placement_style=Triangular  block_type=mult
  rere : xbsIndex_r4/Mult  precision=Full  arith_type="Signed  (2's comp)"  n_bits=16  bin_pt=14  quantization=Truncate  overflow=Wrap  en=off  latency=1  dbl_ovrd=off  use_behavioral_HDL=off  opt=Speed  use_embedded=on  optimum_pipeline=off  pipeline=on  use_rpm=on  placement_style=Triangular  block_type=mult
  ri_to_c : casper_library_misc/ri_to_c
  ab : Outport
  wires:
  ri_to_c/1 -> ab/1
  convert_im/1 -> ri_to_c/2
  convert_re/1 -> ri_to_c/1
  addsub_im/1 -> convert_im/1
  addsub_re/1 -> convert_re/1
  reim/1 -> addsub_im/2
  imre/1 -> addsub_im/1
  imim/1 -> addsub_re/2
  rere/1 -> addsub_re/1
  b_expand/4(lsb_out1) -> reim/2
  a_expand/3(out2) -> reim/1
  b_expand/3(out2) -> imre/2
  a_expand/4(lsb_out1) -> imre/1
  b_expand/2(out3) -> imim/2
  a_expand/2(out3) -> imim/1
  b_expand/1(msb_out4) -> rere/2
  a_expand/1(msb_out4) -> rere/1
  b_replicate/1(out) -> b_expand/1(bus_in)
  a_replicate/1(out) -> a_expand/1(bus_in)
  b/1 -> b_replicate/1(in)
  a/1 -> a_replicate/1(in)

== system casper_library_correlator/auto_tap/dual_pol_cmac/cmac3/ri_to_c ==
  In1 : Inport
  In2 : Inport  Port=2
  Concat : xbsIndex_r4/Concat  num_inputs=2  dbl_ovrd=off  block_type=concat
      settings: block_version=9.2.01
  Reinterpret : xbsIndex_r4/Reinterpret  force_arith_type=on  arith_type=Unsigned  force_bin_pt=on  bin_pt=0  block_type=reinterpret
      settings: infoedit="Changes signal type without altering the binary representation.   You can changed the signal between signed and unsigned, and relocate the binary point.<P><P>Hardware notes: In hardware this block costs nothing.<P><P>Example:  Suppose the input is 6 bits wide, signed, with 2 fractional bits, and the output is forced to unsigned with 0 fractional bits.  Then an input of -2.0 (1110.00 in binary 2's complement) becomes an output of 56 (111000 in binary)."  block_version=9.2.01
  Reinterpret1 : xbsIndex_r4/Reinterpret  force_arith_type=on  arith_type=Unsigned  force_bin_pt=on  bin_pt=0  block_type=reinterpret
      settings: infoedit="Changes signal type without altering the binary representation.   You can changed the signal between signed and unsigned, and relocate the binary point.<P><P>Hardware notes: In hardware this block costs nothing.<P><P>Example:  Suppose the input is 6 bits wide, signed, with 2 fractional bits, and the output is forced to unsigned with 0 fractional bits.  Then an input of -2.0 (1110.00 in binary 2's complement) becomes an output of 56 (111000 in binary)."  block_version=9.2.01
  Out1 : Outport
  wires:
  In2/1 -> Reinterpret1/1
  Concat/1 -> Out1/1
  In1/1 -> Reinterpret/1
  Reinterpret1/1 -> Concat/2
  Reinterpret/1 -> Concat/1
